simulink model "pfb_fft_d3a"  (R2021a)
settings: Solver=VariableStepAuto  StartTime=0.0  StopTime=100.0  RelTol=1e-3
undefined symbols (not defined in the file): i, pfb_coeff_gen_calc
libraries: xbsIndex_r4 x11529, casper_library_misc x39, casper_library_delays x39, xbsReplacements_r4 x2
(part 2 of 118)

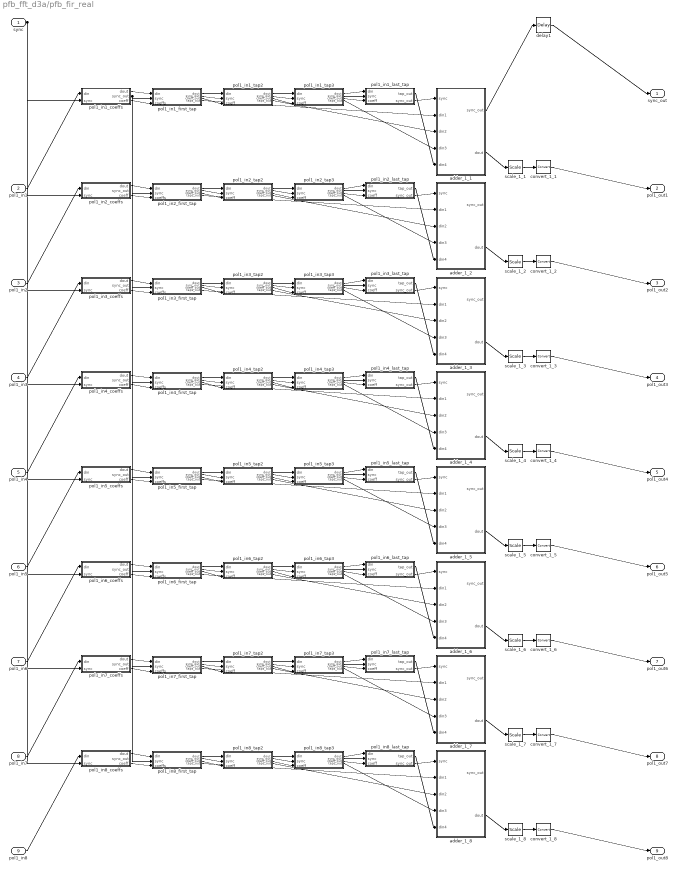
== system pfb_fft_d3a/pfb_fir_real ==
  sync : Inport
  pol1_in1 : Inport  Port=2
  pol1_in2 : Inport  Port=3
  pol1_in3 : Inport  Port=4
  pol1_in4 : Inport  Port=5
  pol1_in5 : Inport  Port=6
  pol1_in6 : Inport  Port=7
  pol1_in7 : Inport  Port=8
  pol1_in8 : Inport  Port=9
  adder_1_1 : Subsystem  AncestorBlock=casper_library_misc/adder_tree  mask(adder_tree){n_inputs=4, csp_latency=1, adder_imp=Fabric, first_stage_hdl=on, floating_point=off, dvalid_en=off, float_type=single, frac_width=0, exp_width=0}
      mask prompts: n_inputs "Number of Inputs"; csp_latency "Add Latency"; adder_imp "Adder implementation"; first_stage_hdl "Use behavioural HDL for first stage of adders"; floating_point "floating point"; float_type "float type"; frac_width "fraction length"; exp_width "exponent length"
      mask help:
      | Sums all inputs using a tree of adds and delays.
      |
      | Number of inputs: The number of inputs to the block to be summed
      | Add latency: The number of clock cycles to perform one addition (affects timing)..
      | Adder implementation: choice of fabric or DSP48E core, or behavioral HDL
      | Use behavioural HDL for first stage of adders: Causes the first stage of adders to be absorbed into DSP blocks if multipliers precede them (Virtex 5). Overrides Adder implementation
      mask init:
      | adder_tree_init(gcb, ...
      |     'n_inputs', n_inputs, ...
      |     'csp_latency', csp_latency, ...
      |     'adder_imp', adder_imp, ...
      |     'dvalid_en', dvalid_en, ...
      |     'floating_point', floating_point, ...
      |     'float_type', float_type, ...
      |     'exp_width', exp_width, ...
      |     'frac_width', frac_width, ...     
      |     'first_stage_hdl', first_stage_hdl);
      settings: AttributesFormatString=latency 2
      mask Help: eval('xlWeb(''http://casper.berkeley.edu/wiki/Adder_tree'')')
      mask TypeOptions adder_imp: Behavioral | Fabric | DSP48
      mask Callback floating_point:
      | onoff = get_param(gcb, 'floating_point');
      | if strcmp(onoff,'on')
      |     enable_fixpt = 'off';
      |     set_param_state(gcb, 'float_type', 'on')
      | 
      |     f_type = get_param(gcb, 'float_type');
      |     if strcmp(f_type,'custom')
      |         set_param_state(gcb, 'exp_width', 'on')
      |         set_param_state(gcb, 'frac_width', 'on')
      |     else
      |         set_param_state(gcb, 'exp_width', 'off')
      |         set_param_state(gcb, 'frac_width', 'off')
      |     end
      | 
      | 
      | else
      |     enable_fixpt = 'on';
      |     set_param_state(gcb, 'float_type', 'off')
      |     set_param_state(gcb, 'exp_width', 'off')
      |     set_param_state(gcb, 'frac_width', 'off')
      | end
      mask TypeOptions float_type: single | custom
      mask Callback float_type:
      | f_type = get_param(gcb, 'float_type');
      | if strcmp(f_type,'custom')
      |     set_param_state(gcb, 'exp_width', 'on')
      |     set_param_state(gcb, 'frac_width', 'on')
      | else
      |     set_param_state(gcb, 'exp_width', 'off')
      |     set_param_state(gcb, 'frac_width', 'off')
      | end
  adder_1_2 : Subsystem  AncestorBlock=casper_library_misc/adder_tree  mask(adder_tree){n_inputs=4, csp_latency=1, adder_imp=Fabric, first_stage_hdl=on, floating_point=off, dvalid_en=off, float_type=single, frac_width=0, exp_width=0}
      mask prompts: n_inputs "Number of Inputs"; csp_latency "Add Latency"; adder_imp "Adder implementation"; first_stage_hdl "Use behavioural HDL for first stage of adders"; floating_point "floating point"; float_type "float type"; frac_width "fraction length"; exp_width "exponent length"
      mask help:
      | Sums all inputs using a tree of adds and delays.
      |
      | Number of inputs: The number of inputs to the block to be summed
      | Add latency: The number of clock cycles to perform one addition (affects timing)..
      | Adder implementation: choice of fabric or DSP48E core, or behavioral HDL
      | Use behavioural HDL for first stage of adders: Causes the first stage of adders to be absorbed into DSP blocks if multipliers precede them (Virtex 5). Overrides Adder implementation
      mask init: same as pfb_fft_d3a/pfb_fir_real/adder_1_1
      settings: AttributesFormatString=latency 2
      mask Help: eval('xlWeb(''http://casper.berkeley.edu/wiki/Adder_tree'')')
      mask TypeOptions adder_imp: Behavioral | Fabric | DSP48
      mask Callback floating_point:
      | onoff = get_param(gcb, 'floating_point');
      | if strcmp(onoff,'on')
      |     enable_fixpt = 'off';
      |     set_param_state(gcb, 'float_type', 'on')
      | 
      |     f_type = get_param(gcb, 'float_type');
      |     if strcmp(f_type,'custom')
      |         set_param_state(gcb, 'exp_width', 'on')
      |         set_param_state(gcb, 'frac_width', 'on')
      |     else
      |         set_param_state(gcb, 'exp_width', 'off')
      |         set_param_state(gcb, 'frac_width', 'off')
      |     end
      | 
      | 
      | else
      |     enable_fixpt = 'on';
      |     set_param_state(gcb, 'float_type', 'off')
      |     set_param_state(gcb, 'exp_width', 'off')
      |     set_param_state(gcb, 'frac_width', 'off')
      | end
      mask TypeOptions float_type: single | custom
      mask Callback float_type:
      | f_type = get_param(gcb, 'float_type');
      | if strcmp(f_type,'custom')
      |     set_param_state(gcb, 'exp_width', 'on')
      |     set_param_state(gcb, 'frac_width', 'on')
      | else
      |     set_param_state(gcb, 'exp_width', 'off')
      |     set_param_state(gcb, 'frac_width', 'off')
      | end
  adder_1_3 : Subsystem  AncestorBlock=casper_library_misc/adder_tree  mask(adder_tree){n_inputs=4, csp_latency=1, adder_imp=Fabric, first_stage_hdl=on, floating_point=off, dvalid_en=off, float_type=single, frac_width=0, exp_width=0}
      mask prompts: n_inputs "Number of Inputs"; csp_latency "Add Latency"; adder_imp "Adder implementation"; first_stage_hdl "Use behavioural HDL for first stage of adders"; floating_point "floating point"; float_type "float type"; frac_width "fraction length"; exp_width "exponent length"
      mask help:
      | Sums all inputs using a tree of adds and delays.
      |
      | Number of inputs: The number of inputs to the block to be summed
      | Add latency: The number of clock cycles to perform one addition (affects timing)..
      | Adder implementation: choice of fabric or DSP48E core, or behavioral HDL
      | Use behavioural HDL for first stage of adders: Causes the first stage of adders to be absorbed into DSP blocks if multipliers precede them (Virtex 5). Overrides Adder implementation
      mask init: same as pfb_fft_d3a/pfb_fir_real/adder_1_1
      settings: AttributesFormatString=latency 2
      mask Help: eval('xlWeb(''http://casper.berkeley.edu/wiki/Adder_tree'')')
      mask TypeOptions adder_imp: Behavioral | Fabric | DSP48
      mask Callback floating_point:
      | onoff = get_param(gcb, 'floating_point');
      | if strcmp(onoff,'on')
      |     enable_fixpt = 'off';
      |     set_param_state(gcb, 'float_type', 'on')
      | 
      |     f_type = get_param(gcb, 'float_type');
      |     if strcmp(f_type,'custom')
      |         set_param_state(gcb, 'exp_width', 'on')
      |         set_param_state(gcb, 'frac_width', 'on')
      |     else
      |         set_param_state(gcb, 'exp_width', 'off')
      |         set_param_state(gcb, 'frac_width', 'off')
      |     end
      | 
      | 
      | else
      |     enable_fixpt = 'on';
      |     set_param_state(gcb, 'float_type', 'off')
      |     set_param_state(gcb, 'exp_width', 'off')
      |     set_param_state(gcb, 'frac_width', 'off')
      | end
      mask TypeOptions float_type: single | custom
      mask Callback float_type:
      | f_type = get_param(gcb, 'float_type');
      | if strcmp(f_type,'custom')
      |     set_param_state(gcb, 'exp_width', 'on')
      |     set_param_state(gcb, 'frac_width', 'on')
      | else
      |     set_param_state(gcb, 'exp_width', 'off')
      |     set_param_state(gcb, 'frac_width', 'off')
      | end
  adder_1_4 : Subsystem  AncestorBlock=casper_library_misc/adder_tree  mask(adder_tree){n_inputs=4, csp_latency=1, adder_imp=Fabric, first_stage_hdl=on, floating_point=off, dvalid_en=off, float_type=single, frac_width=0, exp_width=0}
      mask prompts: n_inputs "Number of Inputs"; csp_latency "Add Latency"; adder_imp "Adder implementation"; first_stage_hdl "Use behavioural HDL for first stage of adders"; floating_point "floating point"; float_type "float type"; frac_width "fraction length"; exp_width "exponent length"
      mask help:
      | Sums all inputs using a tree of adds and delays.
      |
      | Number of inputs: The number of inputs to the block to be summed
      | Add latency: The number of clock cycles to perform one addition (affects timing)..
      | Adder implementation: choice of fabric or DSP48E core, or behavioral HDL
      | Use behavioural HDL for first stage of adders: Causes the first stage of adders to be absorbed into DSP blocks if multipliers precede them (Virtex 5). Overrides Adder implementation
      mask init: same as pfb_fft_d3a/pfb_fir_real/adder_1_1
      settings: AttributesFormatString=latency 2
      mask Help: eval('xlWeb(''http://casper.berkeley.edu/wiki/Adder_tree'')')
      mask TypeOptions adder_imp: Behavioral | Fabric | DSP48
      mask Callback floating_point:
      | onoff = get_param(gcb, 'floating_point');
      | if strcmp(onoff,'on')
      |     enable_fixpt = 'off';
      |     set_param_state(gcb, 'float_type', 'on')
      | 
      |     f_type = get_param(gcb, 'float_type');
      |     if strcmp(f_type,'custom')
      |         set_param_state(gcb, 'exp_width', 'on')
      |         set_param_state(gcb, 'frac_width', 'on')
      |     else
      |         set_param_state(gcb, 'exp_width', 'off')
      |         set_param_state(gcb, 'frac_width', 'off')
      |     end
      | 
      | 
      | else
      |     enable_fixpt = 'on';
      |     set_param_state(gcb, 'float_type', 'off')
      |     set_param_state(gcb, 'exp_width', 'off')
      |     set_param_state(gcb, 'frac_width', 'off')
      | end
      mask TypeOptions float_type: single | custom
      mask Callback float_type:
      | f_type = get_param(gcb, 'float_type');
      | if strcmp(f_type,'custom')
      |     set_param_state(gcb, 'exp_width', 'on')
      |     set_param_state(gcb, 'frac_width', 'on')
      | else
      |     set_param_state(gcb, 'exp_width', 'off')
      |     set_param_state(gcb, 'frac_width', 'off')
      | end
  adder_1_5 : Subsystem  AncestorBlock=casper_library_misc/adder_tree  mask(adder_tree){n_inputs=4, csp_latency=1, adder_imp=Fabric, first_stage_hdl=on, floating_point=off, dvalid_en=off, float_type=single, frac_width=0, exp_width=0}
      mask prompts: n_inputs "Number of Inputs"; csp_latency "Add Latency"; adder_imp "Adder implementation"; first_stage_hdl "Use behavioural HDL for first stage of adders"; floating_point "floating point"; float_type "float type"; frac_width "fraction length"; exp_width "exponent length"
      mask help:
      | Sums all inputs using a tree of adds and delays.
      |
      | Number of inputs: The number of inputs to the block to be summed
      | Add latency: The number of clock cycles to perform one addition (affects timing)..
      | Adder implementation: choice of fabric or DSP48E core, or behavioral HDL
      | Use behavioural HDL for first stage of adders: Causes the first stage of adders to be absorbed into DSP blocks if multipliers precede them (Virtex 5). Overrides Adder implementation
      mask init: same as pfb_fft_d3a/pfb_fir_real/adder_1_1
      settings: AttributesFormatString=latency 2
      mask Help: eval('xlWeb(''http://casper.berkeley.edu/wiki/Adder_tree'')')
      mask TypeOptions adder_imp: Behavioral | Fabric | DSP48
      mask Callback floating_point:
      | onoff = get_param(gcb, 'floating_point');
      | if strcmp(onoff,'on')
      |     enable_fixpt = 'off';
      |     set_param_state(gcb, 'float_type', 'on')
      | 
      |     f_type = get_param(gcb, 'float_type');
      |     if strcmp(f_type,'custom')
      |         set_param_state(gcb, 'exp_width', 'on')
      |         set_param_state(gcb, 'frac_width', 'on')
      |     else
      |         set_param_state(gcb, 'exp_width', 'off')
      |         set_param_state(gcb, 'frac_width', 'off')
      |     end
      | 
      | 
      | else
      |     enable_fixpt = 'on';
      |     set_param_state(gcb, 'float_type', 'off')
      |     set_param_state(gcb, 'exp_width', 'off')
      |     set_param_state(gcb, 'frac_width', 'off')
      | end
      mask TypeOptions float_type: single | custom
      mask Callback float_type:
      | f_type = get_param(gcb, 'float_type');
      | if strcmp(f_type,'custom')
      |     set_param_state(gcb, 'exp_width', 'on')
      |     set_param_state(gcb, 'frac_width', 'on')
      | else
      |     set_param_state(gcb, 'exp_width', 'off')
      |     set_param_state(gcb, 'frac_width', 'off')
      | end
  adder_1_6 : Subsystem  AncestorBlock=casper_library_misc/adder_tree  mask(adder_tree){n_inputs=4, csp_latency=1, adder_imp=Fabric, first_stage_hdl=on, floating_point=off, dvalid_en=off, float_type=single, frac_width=0, exp_width=0}
      mask prompts: n_inputs "Number of Inputs"; csp_latency "Add Latency"; adder_imp "Adder implementation"; first_stage_hdl "Use behavioural HDL for first stage of adders"; floating_point "floating point"; float_type "float type"; frac_width "fraction length"; exp_width "exponent length"
      mask help:
      | Sums all inputs using a tree of adds and delays.
      |
      | Number of inputs: The number of inputs to the block to be summed
      | Add latency: The number of clock cycles to perform one addition (affects timing)..
      | Adder implementation: choice of fabric or DSP48E core, or behavioral HDL
      | Use behavioural HDL for first stage of adders: Causes the first stage of adders to be absorbed into DSP blocks if multipliers precede them (Virtex 5). Overrides Adder implementation
      mask init: same as pfb_fft_d3a/pfb_fir_real/adder_1_1
      settings: AttributesFormatString=latency 2
      mask Help: eval('xlWeb(''http://casper.berkeley.edu/wiki/Adder_tree'')')
      mask TypeOptions adder_imp: Behavioral | Fabric | DSP48
      mask Callback floating_point:
      | onoff = get_param(gcb, 'floating_point');
      | if strcmp(onoff,'on')
      |     enable_fixpt = 'off';
      |     set_param_state(gcb, 'float_type', 'on')
      | 
      |     f_type = get_param(gcb, 'float_type');
      |     if strcmp(f_type,'custom')
      |         set_param_state(gcb, 'exp_width', 'on')
      |         set_param_state(gcb, 'frac_width', 'on')
      |     else
      |         set_param_state(gcb, 'exp_width', 'off')
      |         set_param_state(gcb, 'frac_width', 'off')
      |     end
      | 
      | 
      | else
      |     enable_fixpt = 'on';
      |     set_param_state(gcb, 'float_type', 'off')
      |     set_param_state(gcb, 'exp_width', 'off')
      |     set_param_state(gcb, 'frac_width', 'off')
      | end
      mask TypeOptions float_type: single | custom
      mask Callback float_type:
      | f_type = get_param(gcb, 'float_type');
      | if strcmp(f_type,'custom')
      |     set_param_state(gcb, 'exp_width', 'on')
      |     set_param_state(gcb, 'frac_width', 'on')
      | else
      |     set_param_state(gcb, 'exp_width', 'off')
      |     set_param_state(gcb, 'frac_width', 'off')
      | end
  adder_1_7 : Subsystem  AncestorBlock=casper_library_misc/adder_tree  mask(adder_tree){n_inputs=4, csp_latency=1, adder_imp=Fabric, first_stage_hdl=on, floating_point=off, dvalid_en=off, float_type=single, frac_width=0, exp_width=0}
      mask prompts: n_inputs "Number of Inputs"; csp_latency "Add Latency"; adder_imp "Adder implementation"; first_stage_hdl "Use behavioural HDL for first stage of adders"; floating_point "floating point"; float_type "float type"; frac_width "fraction length"; exp_width "exponent length"
      mask help:
      | Sums all inputs using a tree of adds and delays.
      |
      | Number of inputs: The number of inputs to the block to be summed
      | Add latency: The number of clock cycles to perform one addition (affects timing)..
      | Adder implementation: choice of fabric or DSP48E core, or behavioral HDL
      | Use behavioural HDL for first stage of adders: Causes the first stage of adders to be absorbed into DSP blocks if multipliers precede them (Virtex 5). Overrides Adder implementation
      mask init: same as pfb_fft_d3a/pfb_fir_real/adder_1_1
      settings: AttributesFormatString=latency 2
      mask Help: eval('xlWeb(''http://casper.berkeley.edu/wiki/Adder_tree'')')
      mask TypeOptions adder_imp: Behavioral | Fabric | DSP48
      mask Callback floating_point:
      | onoff = get_param(gcb, 'floating_point');
      | if strcmp(onoff,'on')
      |     enable_fixpt = 'off';
      |     set_param_state(gcb, 'float_type', 'on')
      | 
      |     f_type = get_param(gcb, 'float_type');
      |     if strcmp(f_type,'custom')
      |         set_param_state(gcb, 'exp_width', 'on')
      |         set_param_state(gcb, 'frac_width', 'on')
      |     else
      |         set_param_state(gcb, 'exp_width', 'off')
      |         set_param_state(gcb, 'frac_width', 'off')
      |     end
      | 
      | 
      | else
      |     enable_fixpt = 'on';
      |     set_param_state(gcb, 'float_type', 'off')
      |     set_param_state(gcb, 'exp_width', 'off')
      |     set_param_state(gcb, 'frac_width', 'off')
      | end
      mask TypeOptions float_type: single | custom
      mask Callback float_type:
      | f_type = get_param(gcb, 'float_type');
      | if strcmp(f_type,'custom')
      |     set_param_state(gcb, 'exp_width', 'on')
      |     set_param_state(gcb, 'frac_width', 'on')
      | else
      |     set_param_state(gcb, 'exp_width', 'off')
      |     set_param_state(gcb, 'frac_width', 'off')
      | end
  adder_1_8 : Subsystem  AncestorBlock=casper_library_misc/adder_tree  mask(adder_tree){n_inputs=4, csp_latency=1, adder_imp=Fabric, first_stage_hdl=on, floating_point=off, dvalid_en=off, float_type=single, frac_width=0, exp_width=0}
      mask prompts: n_inputs "Number of Inputs"; csp_latency "Add Latency"; adder_imp "Adder implementation"; first_stage_hdl "Use behavioural HDL for first stage of adders"; floating_point "floating point"; float_type "float type"; frac_width "fraction length"; exp_width "exponent length"
      mask help:
      | Sums all inputs using a tree of adds and delays.
      |
      | Number of inputs: The number of inputs to the block to be summed
      | Add latency: The number of clock cycles to perform one addition (affects timing)..
      | Adder implementation: choice of fabric or DSP48E core, or behavioral HDL
      | Use behavioural HDL for first stage of adders: Causes the first stage of adders to be absorbed into DSP blocks if multipliers precede them (Virtex 5). Overrides Adder implementation
      mask init: same as pfb_fft_d3a/pfb_fir_real/adder_1_1
      settings: AttributesFormatString=latency 2
      mask Help: eval('xlWeb(''http://casper.berkeley.edu/wiki/Adder_tree'')')
      mask TypeOptions adder_imp: Behavioral | Fabric | DSP48
      mask Callback floating_point:
      | onoff = get_param(gcb, 'floating_point');
      | if strcmp(onoff,'on')
      |     enable_fixpt = 'off';
      |     set_param_state(gcb, 'float_type', 'on')
      | 
      |     f_type = get_param(gcb, 'float_type');
      |     if strcmp(f_type,'custom')
      |         set_param_state(gcb, 'exp_width', 'on')
      |         set_param_state(gcb, 'frac_width', 'on')
      |     else
      |         set_param_state(gcb, 'exp_width', 'off')
      |         set_param_state(gcb, 'frac_width', 'off')
      |     end
      | 
      | 
      | else
      |     enable_fixpt = 'on';
      |     set_param_state(gcb, 'float_type', 'off')
      |     set_param_state(gcb, 'exp_width', 'off')
      |     set_param_state(gcb, 'frac_width', 'off')
      | end
      mask TypeOptions float_type: single | custom
      mask Callback float_type:
      | f_type = get_param(gcb, 'float_type');
      | if strcmp(f_type,'custom')
      |     set_param_state(gcb, 'exp_width', 'on')
      |     set_param_state(gcb, 'frac_width', 'on')
      | else
      |     set_param_state(gcb, 'exp_width', 'off')
      |     set_param_state(gcb, 'frac_width', 'off')
      | end
  convert_1_{1..8} (8 alike) : xbsIndex_r4/Convert  gui_display_data_type=Fixed-point  arith_type="Signed  (2's comp)"  n_bits=18  bin_pt=17  float_type=Single  exp_bits=8  fraction_bits=24  quantization="Round  (unbiased: Even Values)"  overflow=Wrap  en=off  latency=1  pipeline=on  dbl_ovrd=off  block_type=convert
  delay1 : xbsIndex_r4/Delay  rst=off  infoeditControl=Selection of Reset will increase slice count due to use of real FFs and instead of SRLs  en=off  latency=1  reg_retiming=off  dbl_ovrd=off  block_type=delay
  pol1_in1_coeffs : Subsystem  AncestorBlock=casper_library_pfbs/pfb_coeff_gen  mask(pfb_coeff_gen){PFBSize=14, CoeffBitWidth=18, TotalTaps=4, CoeffDistMem=off, WindowType=hamming, bram_latency=2, n_inputs=3, nput=0, fwidth=1, debug_mode=off, fan_latency=1}
      mask prompts: PFBSize "Size of PFB: (2^? pnts)"; CoeffBitWidth "Bitwidth of Coefficients:"; TotalTaps "Total Number of Taps:"; CoeffDistMem "Implement Coeff Gen in Distributed Memory"; WindowType "Windowing Function:"; bram_latency "BRAM Latency"; n_inputs "Number of Simultaneous Inputs: (2^?)"; nput "This is input number:"; fwidth "Bin Width (normal=1)"; debug_mode "Debug mode - coeffs are a [1:pfb_size*taps] ramp."; fan_latency "Fanout latency"
      mask init:
      | pfb_coeff_gen_init(gcb, ...
      |     'PFBSize', PFBSize, ...
      |     'CoeffBitWidth', CoeffBitWidth, ...
      |     'TotalTaps', TotalTaps, ...
      |     'CoeffDistMem', CoeffDistMem, ...
      |     'WindowType', WindowType, ...
      |     'bram_latency', bram_latency, ...
      |     'n_inputs', n_inputs, ...
      |     'nput', nput, ...
      |     'fwidth', fwidth, ...
      |     'fan_latency', fan_latency, ...
      |     'debug_mode', debug_mode);
      settings: AttributesFormatString=|
      | PFBSize=14, n_inputs=3,
      | taps=4, input=0
  pol1_in1_first_tap : Subsystem  AncestorBlock=casper_library_pfbs/first_tap_real  mask(first_tap_real){PFBSize=14, n_pol_blocks=1, CoeffBitWidth=18, TotalTaps=4, BitWidthIn=14, WindowType=hamming, mult_latency=2, bram_latency=2, n_inputs=3, fwidth=1, use_hdl=on, use_embedded=off}
      mask prompts: PFBSize "Size of PFB: (2^? pnts)"; n_pol_blocks "Number of serial polarization blocks"; CoeffBitWidth "Bitwidth of Coefficients:"; TotalTaps "Total Number of Taps:"; BitWidthIn "Input Bitwidth:"; WindowType "Windowing Function:"; mult_latency "Mult Latency"; bram_latency "BRAM Latency"; n_inputs "Number of Simultaneous Inputs: (2^?)"; fwidth "Bit Width (normal=1)"; use_hdl "Use behavioral HDL for multlipliers"; use_embedded "Use embedded multipliers"
      mask init:
      | first_tap_real_init(gcb,...
      |     'PFBSize', PFBSize,...
      |     'CoeffBitWidth', CoeffBitWidth,...
      |     'TotalTaps', TotalTaps,...
      |     'BitWidthIn', BitWidthIn,...
      |     'WindowType', WindowType,...
      |     'mult_latency', mult_latency,...
      |     'bram_latency', bram_latency,...
      |     'n_inputs', n_inputs,...
      |     'n_pol_blocks', n_pol_blocks, ...
      |     'fwidth', fwidth,...
      |     'use_hdl', use_hdl,...
      |     'use_embedded', use_embedded);
      settings: AttributesFormatString=taps=4
      mask TypeOptions WindowType: bartlett | barthannwin | blackman | blackmanharris | bohamwin | chebwin | flattopwin | gausswin | hamming | hann | kaiser | nuttallwin | parzenwin | rectwin | tukeywin | triang | userwindow
      mask Callback use_hdl:
      | use_hdl = get_param(gcb,'use_hdl');
      | if( strcmp(use_hdl,'on')),
      |     set_param(gcb, 'use_embedded','off');
      |     set_param(gcb, 'MaskVisibilities',{'on','on','on','on','on','on','on','on','on','on','on','off'});
      | else,
      |     set_param(gcb, 'MaskVisibilities',{'on','on','on','on','on','on','on','on','on','on','on','on'});
      | end
  pol1_in1_last_tap : Subsystem  AncestorBlock=casper_library_pfbs/last_tap_real  mask(last_tap_real){BitWidthIn=14, CoeffBitWidth=18, mult_latency=2, use_hdl=on, use_embedded=off}
      mask prompts: BitWidthIn "Input Bitwidth:"; CoeffBitWidth "Coeff Bitwidth:"; mult_latency "Mult Latency"; use_hdl "Use behavioral HDL for multlipliers"; use_embedded "Use embedded multipliers"
      mask init:
      | last_tap_real_init(gcb,...
      |     'BitWidthIn', BitWidthIn,...
      |     'CoeffBitWidth', CoeffBitWidth,...
      |     'mult_latency', mult_latency,...
      |     'use_hdl', use_hdl,...
      |     'use_embedded', use_embedded);
      mask Callback use_hdl:
      | use_hdl = get_param(gcb,'use_hdl');
      | if( strcmp(use_hdl,'on')),
      |     set_param(gcb, 'use_embedded','off');
      |     set_param(gcb, 'MaskVisibilities',{'on','on','on','on','off'});
      | else,
      |     set_param(gcb, 'MaskVisibilities',{'on','on','on','on','on'});
      | end
  pol1_in1_tap2 : Subsystem  AncestorBlock=casper_library_pfbs/tap_real  mask(pfb_tap_real){mult_latency=2, coeff_width=18, coeff_frac_width=17, delay=2048, data_width=14, bram_latency=2, use_hdl=on, use_embedded=off}
      mask prompts: mult_latency "Multiplier Latency"; coeff_width "Coefficient Bit Width In"; coeff_frac_width "Coefficient Fractional Bits"; delay "Data/Sync Delay"; data_width "Data Bit Width In"; bram_latency "BRAM Latency"; use_hdl "Use behavioral HDL for multlipliers"; use_embedded "Use embedded multipliers"
      mask init:
      | use_hdl = get_param(gcb,'use_hdl');
      | use_embedded = get_param(gcb,'use_embedded');
      | set_param(gcb,'LinkStatus','inactive');
      | 
      | set_param([gcb,'/Mult'],'use_embedded',use_embedded);
      | set_param([gcb,'/Mult'],'use_behavioral_HDL',use_hdl);
  pol1_in1_tap3 : Subsystem  AncestorBlock=casper_library_pfbs/tap_real  mask(pfb_tap_real){mult_latency=2, coeff_width=18, coeff_frac_width=17, delay=2048, data_width=14, bram_latency=2, use_hdl=on, use_embedded=off}
      mask prompts: mult_latency "Multiplier Latency"; coeff_width "Coefficient Bit Width In"; coeff_frac_width "Coefficient Fractional Bits"; delay "Data/Sync Delay"; data_width "Data Bit Width In"; bram_latency "BRAM Latency"; use_hdl "Use behavioral HDL for multlipliers"; use_embedded "Use embedded multipliers"
      mask init: same as pfb_fft_d3a/pfb_fir_real/pol1_in1_tap2
  pol1_in2_coeffs : Subsystem  AncestorBlock=casper_library_pfbs/pfb_coeff_gen  mask(pfb_coeff_gen){PFBSize=14, CoeffBitWidth=18, TotalTaps=4, CoeffDistMem=off, WindowType=hamming, bram_latency=2, n_inputs=3, nput=1, fwidth=1, debug_mode=off, fan_latency=1}
      mask prompts: PFBSize "Size of PFB: (2^? pnts)"; CoeffBitWidth "Bitwidth of Coefficients:"; TotalTaps "Total Number of Taps:"; CoeffDistMem "Implement Coeff Gen in Distributed Memory"; WindowType "Windowing Function:"; bram_latency "BRAM Latency"; n_inputs "Number of Simultaneous Inputs: (2^?)"; nput "This is input number:"; fwidth "Bin Width (normal=1)"; debug_mode "Debug mode - coeffs are a [1:pfb_size*taps] ramp."; fan_latency "Fanout latency"
      mask init: same as pfb_fft_d3a/pfb_fir_real/pol1_in1_coeffs
      settings: AttributesFormatString=|
      | PFBSize=14, n_inputs=3,
      | taps=4, input=1
  pol1_in2_first_tap : Subsystem  AncestorBlock=casper_library_pfbs/first_tap_real  mask(first_tap_real){PFBSize=14, n_pol_blocks=1, CoeffBitWidth=18, TotalTaps=4, BitWidthIn=14, WindowType=hamming, mult_latency=2, bram_latency=2, n_inputs=3, fwidth=1, use_hdl=on, use_embedded=off}
      mask prompts: PFBSize "Size of PFB: (2^? pnts)"; n_pol_blocks "Number of serial polarization blocks"; CoeffBitWidth "Bitwidth of Coefficients:"; TotalTaps "Total Number of Taps:"; BitWidthIn "Input Bitwidth:"; WindowType "Windowing Function:"; mult_latency "Mult Latency"; bram_latency "BRAM Latency"; n_inputs "Number of Simultaneous Inputs: (2^?)"; fwidth "Bit Width (normal=1)"; use_hdl "Use behavioral HDL for multlipliers"; use_embedded "Use embedded multipliers"
      mask init: same as pfb_fft_d3a/pfb_fir_real/pol1_in1_first_tap
      settings: AttributesFormatString=taps=4
      mask TypeOptions WindowType: bartlett | barthannwin | blackman | blackmanharris | bohamwin | chebwin | flattopwin | gausswin | hamming | hann | kaiser | nuttallwin | parzenwin | rectwin | tukeywin | triang | userwindow
      mask Callback use_hdl:
      | use_hdl = get_param(gcb,'use_hdl');
      | if( strcmp(use_hdl,'on')),
      |     set_param(gcb, 'use_embedded','off');
      |     set_param(gcb, 'MaskVisibilities',{'on','on','on','on','on','on','on','on','on','on','on','off'});
      | else,
      |     set_param(gcb, 'MaskVisibilities',{'on','on','on','on','on','on','on','on','on','on','on','on'});
      | end
  pol1_in2_last_tap : Subsystem  AncestorBlock=casper_library_pfbs/last_tap_real  mask(last_tap_real){BitWidthIn=14, CoeffBitWidth=18, mult_latency=2, use_hdl=on, use_embedded=off}
      mask prompts: BitWidthIn "Input Bitwidth:"; CoeffBitWidth "Coeff Bitwidth:"; mult_latency "Mult Latency"; use_hdl "Use behavioral HDL for multlipliers"; use_embedded "Use embedded multipliers"
      mask init:
      | last_tap_real_init(gcb,...
      |     'BitWidthIn', BitWidthIn,...
      |     'CoeffBitWidth', CoeffBitWidth,...
      |     'mult_latency', mult_latency,...
      |     'use_hdl', use_hdl,...
      |     'use_embedded', use_embedded);
      mask Callback use_hdl:
      | use_hdl = get_param(gcb,'use_hdl');
      | if( strcmp(use_hdl,'on')),
      |     set_param(gcb, 'use_embedded','off');
      |     set_param(gcb, 'MaskVisibilities',{'on','on','on','on','off'});
      | else,
      |     set_param(gcb, 'MaskVisibilities',{'on','on','on','on','on'});
      | end
  pol1_in2_tap2 : Subsystem  AncestorBlock=casper_library_pfbs/tap_real  mask(pfb_tap_real){mult_latency=2, coeff_width=18, coeff_frac_width=17, delay=2048, data_width=14, bram_latency=2, use_hdl=on, use_embedded=off}
      mask prompts: mult_latency "Multiplier Latency"; coeff_width "Coefficient Bit Width In"; coeff_frac_width "Coefficient Fractional Bits"; delay "Data/Sync Delay"; data_width "Data Bit Width In"; bram_latency "BRAM Latency"; use_hdl "Use behavioral HDL for multlipliers"; use_embedded "Use embedded multipliers"
      mask init: same as pfb_fft_d3a/pfb_fir_real/pol1_in1_tap2
  pol1_in2_tap3 : Subsystem  AncestorBlock=casper_library_pfbs/tap_real  mask(pfb_tap_real){mult_latency=2, coeff_width=18, coeff_frac_width=17, delay=2048, data_width=14, bram_latency=2, use_hdl=on, use_embedded=off}
      mask prompts: mult_latency "Multiplier Latency"; coeff_width "Coefficient Bit Width In"; coeff_frac_width "Coefficient Fractional Bits"; delay "Data/Sync Delay"; data_width "Data Bit Width In"; bram_latency "BRAM Latency"; use_hdl "Use behavioral HDL for multlipliers"; use_embedded "Use embedded multipliers"
      mask init: same as pfb_fft_d3a/pfb_fir_real/pol1_in1_tap2
  pol1_in3_coeffs : Subsystem  AncestorBlock=casper_library_pfbs/pfb_coeff_gen  mask(pfb_coeff_gen){PFBSize=14, CoeffBitWidth=18, TotalTaps=4, CoeffDistMem=off, WindowType=hamming, bram_latency=2, n_inputs=3, nput=2, fwidth=1, debug_mode=off, fan_latency=1}
      mask prompts: PFBSize "Size of PFB: (2^? pnts)"; CoeffBitWidth "Bitwidth of Coefficients:"; TotalTaps "Total Number of Taps:"; CoeffDistMem "Implement Coeff Gen in Distributed Memory"; WindowType "Windowing Function:"; bram_latency "BRAM Latency"; n_inputs "Number of Simultaneous Inputs: (2^?)"; nput "This is input number:"; fwidth "Bin Width (normal=1)"; debug_mode "Debug mode - coeffs are a [1:pfb_size*taps] ramp."; fan_latency "Fanout latency"
      mask init: same as pfb_fft_d3a/pfb_fir_real/pol1_in1_coeffs
      settings: AttributesFormatString=|
      | PFBSize=14, n_inputs=3,
      | taps=4, input=2
  pol1_in3_first_tap : Subsystem  AncestorBlock=casper_library_pfbs/first_tap_real  mask(first_tap_real){PFBSize=14, n_pol_blocks=1, CoeffBitWidth=18, TotalTaps=4, BitWidthIn=14, WindowType=hamming, mult_latency=2, bram_latency=2, n_inputs=3, fwidth=1, use_hdl=on, use_embedded=off}
      mask prompts: PFBSize "Size of PFB: (2^? pnts)"; n_pol_blocks "Number of serial polarization blocks"; CoeffBitWidth "Bitwidth of Coefficients:"; TotalTaps "Total Number of Taps:"; BitWidthIn "Input Bitwidth:"; WindowType "Windowing Function:"; mult_latency "Mult Latency"; bram_latency "BRAM Latency"; n_inputs "Number of Simultaneous Inputs: (2^?)"; fwidth "Bit Width (normal=1)"; use_hdl "Use behavioral HDL for multlipliers"; use_embedded "Use embedded multipliers"
      mask init: same as pfb_fft_d3a/pfb_fir_real/pol1_in1_first_tap
      settings: AttributesFormatString=taps=4
      mask TypeOptions WindowType: bartlett | barthannwin | blackman | blackmanharris | bohamwin | chebwin | flattopwin | gausswin | hamming | hann | kaiser | nuttallwin | parzenwin | rectwin | tukeywin | triang | userwindow
      mask Callback use_hdl:
      | use_hdl = get_param(gcb,'use_hdl');
      | if( strcmp(use_hdl,'on')),
      |     set_param(gcb, 'use_embedded','off');
      |     set_param(gcb, 'MaskVisibilities',{'on','on','on','on','on','on','on','on','on','on','on','off'});
      | else,
      |     set_param(gcb, 'MaskVisibilities',{'on','on','on','on','on','on','on','on','on','on','on','on'});
      | end
  pol1_in3_last_tap : Subsystem  AncestorBlock=casper_library_pfbs/last_tap_real  mask(last_tap_real){BitWidthIn=14, CoeffBitWidth=18, mult_latency=2, use_hdl=on, use_embedded=off}
      mask prompts: BitWidthIn "Input Bitwidth:"; CoeffBitWidth "Coeff Bitwidth:"; mult_latency "Mult Latency"; use_hdl "Use behavioral HDL for multlipliers"; use_embedded "Use embedded multipliers"
      mask init:
      | last_tap_real_init(gcb,...
      |     'BitWidthIn', BitWidthIn,...
      |     'CoeffBitWidth', CoeffBitWidth,...
      |     'mult_latency', mult_latency,...
      |     'use_hdl', use_hdl,...
      |     'use_embedded', use_embedded);
      mask Callback use_hdl:
      | use_hdl = get_param(gcb,'use_hdl');
      | if( strcmp(use_hdl,'on')),
      |     set_param(gcb, 'use_embedded','off');
      |     set_param(gcb, 'MaskVisibilities',{'on','on','on','on','off'});
      | else,
      |     set_param(gcb, 'MaskVisibilities',{'on','on','on','on','on'});
      | end
  pol1_in3_tap2 : Subsystem  AncestorBlock=casper_library_pfbs/tap_real  mask(pfb_tap_real){mult_latency=2, coeff_width=18, coeff_frac_width=17, delay=2048, data_width=14, bram_latency=2, use_hdl=on, use_embedded=off}
      mask prompts: mult_latency "Multiplier Latency"; coeff_width "Coefficient Bit Width In"; coeff_frac_width "Coefficient Fractional Bits"; delay "Data/Sync Delay"; data_width "Data Bit Width In"; bram_latency "BRAM Latency"; use_hdl "Use behavioral HDL for multlipliers"; use_embedded "Use embedded multipliers"
      mask init: same as pfb_fft_d3a/pfb_fir_real/pol1_in1_tap2
  pol1_in3_tap3 : Subsystem  AncestorBlock=casper_library_pfbs/tap_real  mask(pfb_tap_real){mult_latency=2, coeff_width=18, coeff_frac_width=17, delay=2048, data_width=14, bram_latency=2, use_hdl=on, use_embedded=off}
      mask prompts: mult_latency "Multiplier Latency"; coeff_width "Coefficient Bit Width In"; coeff_frac_width "Coefficient Fractional Bits"; delay "Data/Sync Delay"; data_width "Data Bit Width In"; bram_latency "BRAM Latency"; use_hdl "Use behavioral HDL for multlipliers"; use_embedded "Use embedded multipliers"
      mask init: same as pfb_fft_d3a/pfb_fir_real/pol1_in1_tap2
  pol1_in4_coeffs : Subsystem  AncestorBlock=casper_library_pfbs/pfb_coeff_gen  mask(pfb_coeff_gen){PFBSize=14, CoeffBitWidth=18, TotalTaps=4, CoeffDistMem=off, WindowType=hamming, bram_latency=2, n_inputs=3, nput=3, fwidth=1, debug_mode=off, fan_latency=1}
      mask prompts: PFBSize "Size of PFB: (2^? pnts)"; CoeffBitWidth "Bitwidth of Coefficients:"; TotalTaps "Total Number of Taps:"; CoeffDistMem "Implement Coeff Gen in Distributed Memory"; WindowType "Windowing Function:"; bram_latency "BRAM Latency"; n_inputs "Number of Simultaneous Inputs: (2^?)"; nput "This is input number:"; fwidth "Bin Width (normal=1)"; debug_mode "Debug mode - coeffs are a [1:pfb_size*taps] ramp."; fan_latency "Fanout latency"
      mask init: same as pfb_fft_d3a/pfb_fir_real/pol1_in1_coeffs
      settings: AttributesFormatString=|
      | PFBSize=14, n_inputs=3,
      | taps=4, input=3
  pol1_in4_first_tap : Subsystem  AncestorBlock=casper_library_pfbs/first_tap_real  mask(first_tap_real){PFBSize=14, n_pol_blocks=1, CoeffBitWidth=18, TotalTaps=4, BitWidthIn=14, WindowType=hamming, mult_latency=2, bram_latency=2, n_inputs=3, fwidth=1, use_hdl=on, use_embedded=off}
      mask prompts: PFBSize "Size of PFB: (2^? pnts)"; n_pol_blocks "Number of serial polarization blocks"; CoeffBitWidth "Bitwidth of Coefficients:"; TotalTaps "Total Number of Taps:"; BitWidthIn "Input Bitwidth:"; WindowType "Windowing Function:"; mult_latency "Mult Latency"; bram_latency "BRAM Latency"; n_inputs "Number of Simultaneous Inputs: (2^?)"; fwidth "Bit Width (normal=1)"; use_hdl "Use behavioral HDL for multlipliers"; use_embedded "Use embedded multipliers"
      mask init: same as pfb_fft_d3a/pfb_fir_real/pol1_in1_first_tap
      settings: AttributesFormatString=taps=4
      mask TypeOptions WindowType: bartlett | barthannwin | blackman | blackmanharris | bohamwin | chebwin | flattopwin | gausswin | hamming | hann | kaiser | nuttallwin | parzenwin | rectwin | tukeywin | triang | userwindow
      mask Callback use_hdl:
      | use_hdl = get_param(gcb,'use_hdl');
      | if( strcmp(use_hdl,'on')),
      |     set_param(gcb, 'use_embedded','off');
      |     set_param(gcb, 'MaskVisibilities',{'on','on','on','on','on','on','on','on','on','on','on','off'});
      | else,
      |     set_param(gcb, 'MaskVisibilities',{'on','on','on','on','on','on','on','on','on','on','on','on'});
      | end
  pol1_in4_last_tap : Subsystem  AncestorBlock=casper_library_pfbs/last_tap_real  mask(last_tap_real){BitWidthIn=14, CoeffBitWidth=18, mult_latency=2, use_hdl=on, use_embedded=off}
      mask prompts: BitWidthIn "Input Bitwidth:"; CoeffBitWidth "Coeff Bitwidth:"; mult_latency "Mult Latency"; use_hdl "Use behavioral HDL for multlipliers"; use_embedded "Use embedded multipliers"
      mask init:
      | last_tap_real_init(gcb,...
      |     'BitWidthIn', BitWidthIn,...
      |     'CoeffBitWidth', CoeffBitWidth,...
      |     'mult_latency', mult_latency,...
      |     'use_hdl', use_hdl,...
      |     'use_embedded', use_embedded);
      mask Callback use_hdl:
      | use_hdl = get_param(gcb,'use_hdl');
      | if( strcmp(use_hdl,'on')),
      |     set_param(gcb, 'use_embedded','off');
      |     set_param(gcb, 'MaskVisibilities',{'on','on','on','on','off'});
      | else,
      |     set_param(gcb, 'MaskVisibilities',{'on','on','on','on','on'});
      | end
  pol1_in4_tap2 : Subsystem  AncestorBlock=casper_library_pfbs/tap_real  mask(pfb_tap_real){mult_latency=2, coeff_width=18, coeff_frac_width=17, delay=2048, data_width=14, bram_latency=2, use_hdl=on, use_embedded=off}
      mask prompts: mult_latency "Multiplier Latency"; coeff_width "Coefficient Bit Width In"; coeff_frac_width "Coefficient Fractional Bits"; delay "Data/Sync Delay"; data_width "Data Bit Width In"; bram_latency "BRAM Latency"; use_hdl "Use behavioral HDL for multlipliers"; use_embedded "Use embedded multipliers"
      mask init: same as pfb_fft_d3a/pfb_fir_real/pol1_in1_tap2
  pol1_in4_tap3 : Subsystem  AncestorBlock=casper_library_pfbs/tap_real  mask(pfb_tap_real){mult_latency=2, coeff_width=18, coeff_frac_width=17, delay=2048, data_width=14, bram_latency=2, use_hdl=on, use_embedded=off}
      mask prompts: mult_latency "Multiplier Latency"; coeff_width "Coefficient Bit Width In"; coeff_frac_width "Coefficient Fractional Bits"; delay "Data/Sync Delay"; data_width "Data Bit Width In"; bram_latency "BRAM Latency"; use_hdl "Use behavioral HDL for multlipliers"; use_embedded "Use embedded multipliers"
      mask init: same as pfb_fft_d3a/pfb_fir_real/pol1_in1_tap2
  pol1_in5_coeffs : Subsystem  AncestorBlock=casper_library_pfbs/pfb_coeff_gen  mask(pfb_coeff_gen){PFBSize=14, CoeffBitWidth=18, TotalTaps=4, CoeffDistMem=off, WindowType=hamming, bram_latency=2, n_inputs=3, nput=4, fwidth=1, debug_mode=off, fan_latency=1}
      mask prompts: PFBSize "Size of PFB: (2^? pnts)"; CoeffBitWidth "Bitwidth of Coefficients:"; TotalTaps "Total Number of Taps:"; CoeffDistMem "Implement Coeff Gen in Distributed Memory"; WindowType "Windowing Function:"; bram_latency "BRAM Latency"; n_inputs "Number of Simultaneous Inputs: (2^?)"; nput "This is input number:"; fwidth "Bin Width (normal=1)"; debug_mode "Debug mode - coeffs are a [1:pfb_size*taps] ramp."; fan_latency "Fanout latency"
      mask init: same as pfb_fft_d3a/pfb_fir_real/pol1_in1_coeffs
      settings: AttributesFormatString=|
      | PFBSize=14, n_inputs=3,
      | taps=4, input=4
  pol1_in5_first_tap : Subsystem  AncestorBlock=casper_library_pfbs/first_tap_real  mask(first_tap_real){PFBSize=14, n_pol_blocks=1, CoeffBitWidth=18, TotalTaps=4, BitWidthIn=14, WindowType=hamming, mult_latency=2, bram_latency=2, n_inputs=3, fwidth=1, use_hdl=on, use_embedded=off}
      mask prompts: PFBSize "Size of PFB: (2^? pnts)"; n_pol_blocks "Number of serial polarization blocks"; CoeffBitWidth "Bitwidth of Coefficients:"; TotalTaps "Total Number of Taps:"; BitWidthIn "Input Bitwidth:"; WindowType "Windowing Function:"; mult_latency "Mult Latency"; bram_latency "BRAM Latency"; n_inputs "Number of Simultaneous Inputs: (2^?)"; fwidth "Bit Width (normal=1)"; use_hdl "Use behavioral HDL for multlipliers"; use_embedded "Use embedded multipliers"
      mask init: same as pfb_fft_d3a/pfb_fir_real/pol1_in1_first_tap
      settings: AttributesFormatString=taps=4
      mask TypeOptions WindowType: bartlett | barthannwin | blackman | blackmanharris | bohamwin | chebwin | flattopwin | gausswin | hamming | hann | kaiser | nuttallwin | parzenwin | rectwin | tukeywin | triang | userwindow
      mask Callback use_hdl:
      | use_hdl = get_param(gcb,'use_hdl');
      | if( strcmp(use_hdl,'on')),
      |     set_param(gcb, 'use_embedded','off');
      |     set_param(gcb, 'MaskVisibilities',{'on','on','on','on','on','on','on','on','on','on','on','off'});
      | else,
      |     set_param(gcb, 'MaskVisibilities',{'on','on','on','on','on','on','on','on','on','on','on','on'});
      | end
  pol1_in5_last_tap : Subsystem  AncestorBlock=casper_library_pfbs/last_tap_real  mask(last_tap_real){BitWidthIn=14, CoeffBitWidth=18, mult_latency=2, use_hdl=on, use_embedded=off}
      mask prompts: BitWidthIn "Input Bitwidth:"; CoeffBitWidth "Coeff Bitwidth:"; mult_latency "Mult Latency"; use_hdl "Use behavioral HDL for multlipliers"; use_embedded "Use embedded multipliers"
      mask init:
      | last_tap_real_init(gcb,...
      |     'BitWidthIn', BitWidthIn,...
      |     'CoeffBitWidth', CoeffBitWidth,...
      |     'mult_latency', mult_latency,...
      |     'use_hdl', use_hdl,...
      |     'use_embedded', use_embedded);
      mask Callback use_hdl:
      | use_hdl = get_param(gcb,'use_hdl');
      | if( strcmp(use_hdl,'on')),
      |     set_param(gcb, 'use_embedded','off');
      |     set_param(gcb, 'MaskVisibilities',{'on','on','on','on','off'});
      | else,
      |     set_param(gcb, 'MaskVisibilities',{'on','on','on','on','on'});
      | end
  pol1_in5_tap2 : Subsystem  AncestorBlock=casper_library_pfbs/tap_real  mask(pfb_tap_real){mult_latency=2, coeff_width=18, coeff_frac_width=17, delay=2048, data_width=14, bram_latency=2, use_hdl=on, use_embedded=off}
      mask prompts: mult_latency "Multiplier Latency"; coeff_width "Coefficient Bit Width In"; coeff_frac_width "Coefficient Fractional Bits"; delay "Data/Sync Delay"; data_width "Data Bit Width In"; bram_latency "BRAM Latency"; use_hdl "Use behavioral HDL for multlipliers"; use_embedded "Use embedded multipliers"
      mask init: same as pfb_fft_d3a/pfb_fir_real/pol1_in1_tap2
  pol1_in5_tap3 : Subsystem  AncestorBlock=casper_library_pfbs/tap_real  mask(pfb_tap_real){mult_latency=2, coeff_width=18, coeff_frac_width=17, delay=2048, data_width=14, bram_latency=2, use_hdl=on, use_embedded=off}
      mask prompts: mult_latency "Multiplier Latency"; coeff_width "Coefficient Bit Width In"; coeff_frac_width "Coefficient Fractional Bits"; delay "Data/Sync Delay"; data_width "Data Bit Width In"; bram_latency "BRAM Latency"; use_hdl "Use behavioral HDL for multlipliers"; use_embedded "Use embedded multipliers"
      mask init: same as pfb_fft_d3a/pfb_fir_real/pol1_in1_tap2
  pol1_in6_coeffs : Subsystem  AncestorBlock=casper_library_pfbs/pfb_coeff_gen  mask(pfb_coeff_gen){PFBSize=14, CoeffBitWidth=18, TotalTaps=4, CoeffDistMem=off, WindowType=hamming, bram_latency=2, n_inputs=3, nput=5, fwidth=1, debug_mode=off, fan_latency=1}
      mask prompts: PFBSize "Size of PFB: (2^? pnts)"; CoeffBitWidth "Bitwidth of Coefficients:"; TotalTaps "Total Number of Taps:"; CoeffDistMem "Implement Coeff Gen in Distributed Memory"; WindowType "Windowing Function:"; bram_latency "BRAM Latency"; n_inputs "Number of Simultaneous Inputs: (2^?)"; nput "This is input number:"; fwidth "Bin Width (normal=1)"; debug_mode "Debug mode - coeffs are a [1:pfb_size*taps] ramp."; fan_latency "Fanout latency"
      mask init: same as pfb_fft_d3a/pfb_fir_real/pol1_in1_coeffs
      settings: AttributesFormatString=|
      | PFBSize=14, n_inputs=3,
      | taps=4, input=5
  pol1_in6_first_tap : Subsystem  AncestorBlock=casper_library_pfbs/first_tap_real  mask(first_tap_real){PFBSize=14, n_pol_blocks=1, CoeffBitWidth=18, TotalTaps=4, BitWidthIn=14, WindowType=hamming, mult_latency=2, bram_latency=2, n_inputs=3, fwidth=1, use_hdl=on, use_embedded=off}
      mask prompts: PFBSize "Size of PFB: (2^? pnts)"; n_pol_blocks "Number of serial polarization blocks"; CoeffBitWidth "Bitwidth of Coefficients:"; TotalTaps "Total Number of Taps:"; BitWidthIn "Input Bitwidth:"; WindowType "Windowing Function:"; mult_latency "Mult Latency"; bram_latency "BRAM Latency"; n_inputs "Number of Simultaneous Inputs: (2^?)"; fwidth "Bit Width (normal=1)"; use_hdl "Use behavioral HDL for multlipliers"; use_embedded "Use embedded multipliers"
      mask init: same as pfb_fft_d3a/pfb_fir_real/pol1_in1_first_tap
      settings: AttributesFormatString=taps=4
      mask TypeOptions WindowType: bartlett | barthannwin | blackman | blackmanharris | bohamwin | chebwin | flattopwin | gausswin | hamming | hann | kaiser | nuttallwin | parzenwin | rectwin | tukeywin | triang | userwindow
      mask Callback use_hdl:
      | use_hdl = get_param(gcb,'use_hdl');
      | if( strcmp(use_hdl,'on')),
      |     set_param(gcb, 'use_embedded','off');
      |     set_param(gcb, 'MaskVisibilities',{'on','on','on','on','on','on','on','on','on','on','on','off'});
      | else,
      |     set_param(gcb, 'MaskVisibilities',{'on','on','on','on','on','on','on','on','on','on','on','on'});
      | end
  pol1_in6_last_tap : Subsystem  AncestorBlock=casper_library_pfbs/last_tap_real  mask(last_tap_real){BitWidthIn=14, CoeffBitWidth=18, mult_latency=2, use_hdl=on, use_embedded=off}
      mask prompts: BitWidthIn "Input Bitwidth:"; CoeffBitWidth "Coeff Bitwidth:"; mult_latency "Mult Latency"; use_hdl "Use behavioral HDL for multlipliers"; use_embedded "Use embedded multipliers"
      mask init:
      | last_tap_real_init(gcb,...
      |     'BitWidthIn', BitWidthIn,...
      |     'CoeffBitWidth', CoeffBitWidth,...
      |     'mult_latency', mult_latency,...
      |     'use_hdl', use_hdl,...
      |     'use_embedded', use_embedded);
      mask Callback use_hdl:
      | use_hdl = get_param(gcb,'use_hdl');
      | if( strcmp(use_hdl,'on')),
      |     set_param(gcb, 'use_embedded','off');
      |     set_param(gcb, 'MaskVisibilities',{'on','on','on','on','off'});
      | else,
      |     set_param(gcb, 'MaskVisibilities',{'on','on','on','on','on'});
      | end
  pol1_in6_tap2 : Subsystem  AncestorBlock=casper_library_pfbs/tap_real  mask(pfb_tap_real){mult_latency=2, coeff_width=18, coeff_frac_width=17, delay=2048, data_width=14, bram_latency=2, use_hdl=on, use_embedded=off}
      mask prompts: mult_latency "Multiplier Latency"; coeff_width "Coefficient Bit Width In"; coeff_frac_width "Coefficient Fractional Bits"; delay "Data/Sync Delay"; data_width "Data Bit Width In"; bram_latency "BRAM Latency"; use_hdl "Use behavioral HDL for multlipliers"; use_embedded "Use embedded multipliers"
      mask init: same as pfb_fft_d3a/pfb_fir_real/pol1_in1_tap2
  pol1_in6_tap3 : Subsystem  AncestorBlock=casper_library_pfbs/tap_real  mask(pfb_tap_real){mult_latency=2, coeff_width=18, coeff_frac_width=17, delay=2048, data_width=14, bram_latency=2, use_hdl=on, use_embedded=off}
      mask prompts: mult_latency "Multiplier Latency"; coeff_width "Coefficient Bit Width In"; coeff_frac_width "Coefficient Fractional Bits"; delay "Data/Sync Delay"; data_width "Data Bit Width In"; bram_latency "BRAM Latency"; use_hdl "Use behavioral HDL for multlipliers"; use_embedded "Use embedded multipliers"
      mask init: same as pfb_fft_d3a/pfb_fir_real/pol1_in1_tap2
  pol1_in7_coeffs : Subsystem  AncestorBlock=casper_library_pfbs/pfb_coeff_gen  mask(pfb_coeff_gen){PFBSize=14, CoeffBitWidth=18, TotalTaps=4, CoeffDistMem=off, WindowType=hamming, bram_latency=2, n_inputs=3, nput=6, fwidth=1, debug_mode=off, fan_latency=1}
      mask prompts: PFBSize "Size of PFB: (2^? pnts)"; CoeffBitWidth "Bitwidth of Coefficients:"; TotalTaps "Total Number of Taps:"; CoeffDistMem "Implement Coeff Gen in Distributed Memory"; WindowType "Windowing Function:"; bram_latency "BRAM Latency"; n_inputs "Number of Simultaneous Inputs: (2^?)"; nput "This is input number:"; fwidth "Bin Width (normal=1)"; debug_mode "Debug mode - coeffs are a [1:pfb_size*taps] ramp."; fan_latency "Fanout latency"
      mask init: same as pfb_fft_d3a/pfb_fir_real/pol1_in1_coeffs
      settings: AttributesFormatString=|
      | PFBSize=14, n_inputs=3,
      | taps=4, input=6
  pol1_in7_first_tap : Subsystem  AncestorBlock=casper_library_pfbs/first_tap_real  mask(first_tap_real){PFBSize=14, n_pol_blocks=1, CoeffBitWidth=18, TotalTaps=4, BitWidthIn=14, WindowType=hamming, mult_latency=2, bram_latency=2, n_inputs=3, fwidth=1, use_hdl=on, use_embedded=off}
      mask prompts: PFBSize "Size of PFB: (2^? pnts)"; n_pol_blocks "Number of serial polarization blocks"; CoeffBitWidth "Bitwidth of Coefficients:"; TotalTaps "Total Number of Taps:"; BitWidthIn "Input Bitwidth:"; WindowType "Windowing Function:"; mult_latency "Mult Latency"; bram_latency "BRAM Latency"; n_inputs "Number of Simultaneous Inputs: (2^?)"; fwidth "Bit Width (normal=1)"; use_hdl "Use behavioral HDL for multlipliers"; use_embedded "Use embedded multipliers"
      mask init: same as pfb_fft_d3a/pfb_fir_real/pol1_in1_first_tap
      settings: AttributesFormatString=taps=4
      mask TypeOptions WindowType: bartlett | barthannwin | blackman | blackmanharris | bohamwin | chebwin | flattopwin | gausswin | hamming | hann | kaiser | nuttallwin | parzenwin | rectwin | tukeywin | triang | userwindow
      mask Callback use_hdl:
      | use_hdl = get_param(gcb,'use_hdl');
      | if( strcmp(use_hdl,'on')),
      |     set_param(gcb, 'use_embedded','off');
      |     set_param(gcb, 'MaskVisibilities',{'on','on','on','on','on','on','on','on','on','on','on','off'});
      | else,
      |     set_param(gcb, 'MaskVisibilities',{'on','on','on','on','on','on','on','on','on','on','on','on'});
      | end
  pol1_in7_last_tap : Subsystem  AncestorBlock=casper_library_pfbs/last_tap_real  mask(last_tap_real){BitWidthIn=14, CoeffBitWidth=18, mult_latency=2, use_hdl=on, use_embedded=off}
      mask prompts: BitWidthIn "Input Bitwidth:"; CoeffBitWidth "Coeff Bitwidth:"; mult_latency "Mult Latency"; use_hdl "Use behavioral HDL for multlipliers"; use_embedded "Use embedded multipliers"
      mask init:
      | last_tap_real_init(gcb,...
      |     'BitWidthIn', BitWidthIn,...
      |     'CoeffBitWidth', CoeffBitWidth,...
      |     'mult_latency', mult_latency,...
      |     'use_hdl', use_hdl,...
      |     'use_embedded', use_embedded);
      mask Callback use_hdl:
      | use_hdl = get_param(gcb,'use_hdl');
      | if( strcmp(use_hdl,'on')),
      |     set_param(gcb, 'use_embedded','off');
      |     set_param(gcb, 'MaskVisibilities',{'on','on','on','on','off'});
      | else,
      |     set_param(gcb, 'MaskVisibilities',{'on','on','on','on','on'});
      | end
  pol1_in7_tap2 : Subsystem  AncestorBlock=casper_library_pfbs/tap_real  mask(pfb_tap_real){mult_latency=2, coeff_width=18, coeff_frac_width=17, delay=2048, data_width=14, bram_latency=2, use_hdl=on, use_embedded=off}
      mask prompts: mult_latency "Multiplier Latency"; coeff_width "Coefficient Bit Width In"; coeff_frac_width "Coefficient Fractional Bits"; delay "Data/Sync Delay"; data_width "Data Bit Width In"; bram_latency "BRAM Latency"; use_hdl "Use behavioral HDL for multlipliers"; use_embedded "Use embedded multipliers"
      mask init: same as pfb_fft_d3a/pfb_fir_real/pol1_in1_tap2
  pol1_in7_tap3 : Subsystem  AncestorBlock=casper_library_pfbs/tap_real  mask(pfb_tap_real){mult_latency=2, coeff_width=18, coeff_frac_width=17, delay=2048, data_width=14, bram_latency=2, use_hdl=on, use_embedded=off}
      mask prompts: mult_latency "Multiplier Latency"; coeff_width "Coefficient Bit Width In"; coeff_frac_width "Coefficient Fractional Bits"; delay "Data/Sync Delay"; data_width "Data Bit Width In"; bram_latency "BRAM Latency"; use_hdl "Use behavioral HDL for multlipliers"; use_embedded "Use embedded multipliers"
      mask init: same as pfb_fft_d3a/pfb_fir_real/pol1_in1_tap2
  pol1_in8_coeffs : Subsystem  AncestorBlock=casper_library_pfbs/pfb_coeff_gen  mask(pfb_coeff_gen){PFBSize=14, CoeffBitWidth=18, TotalTaps=4, CoeffDistMem=off, WindowType=hamming, bram_latency=2, n_inputs=3, nput=7, fwidth=1, debug_mode=off, fan_latency=1}
      mask prompts: PFBSize "Size of PFB: (2^? pnts)"; CoeffBitWidth "Bitwidth of Coefficients:"; TotalTaps "Total Number of Taps:"; CoeffDistMem "Implement Coeff Gen in Distributed Memory"; WindowType "Windowing Function:"; bram_latency "BRAM Latency"; n_inputs "Number of Simultaneous Inputs: (2^?)"; nput "This is input number:"; fwidth "Bin Width (normal=1)"; debug_mode "Debug mode - coeffs are a [1:pfb_size*taps] ramp."; fan_latency "Fanout latency"
      mask init: same as pfb_fft_d3a/pfb_fir_real/pol1_in1_coeffs
      settings: AttributesFormatString=|
      | PFBSize=14, n_inputs=3,
      | taps=4, input=7
  pol1_in8_first_tap : Subsystem  AncestorBlock=casper_library_pfbs/first_tap_real  mask(first_tap_real){PFBSize=14, n_pol_blocks=1, CoeffBitWidth=18, TotalTaps=4, BitWidthIn=14, WindowType=hamming, mult_latency=2, bram_latency=2, n_inputs=3, fwidth=1, use_hdl=on, use_embedded=off}
      mask prompts: PFBSize "Size of PFB: (2^? pnts)"; n_pol_blocks "Number of serial polarization blocks"; CoeffBitWidth "Bitwidth of Coefficients:"; TotalTaps "Total Number of Taps:"; BitWidthIn "Input Bitwidth:"; WindowType "Windowing Function:"; mult_latency "Mult Latency"; bram_latency "BRAM Latency"; n_inputs "Number of Simultaneous Inputs: (2^?)"; fwidth "Bit Width (normal=1)"; use_hdl "Use behavioral HDL for multlipliers"; use_embedded "Use embedded multipliers"
      mask init: same as pfb_fft_d3a/pfb_fir_real/pol1_in1_first_tap
      settings: AttributesFormatString=taps=4
      mask TypeOptions WindowType: bartlett | barthannwin | blackman | blackmanharris | bohamwin | chebwin | flattopwin | gausswin | hamming | hann | kaiser | nuttallwin | parzenwin | rectwin | tukeywin | triang | userwindow
      mask Callback use_hdl:
      | use_hdl = get_param(gcb,'use_hdl');
      | if( strcmp(use_hdl,'on')),
      |     set_param(gcb, 'use_embedded','off');
      |     set_param(gcb, 'MaskVisibilities',{'on','on','on','on','on','on','on','on','on','on','on','off'});
      | else,
      |     set_param(gcb, 'MaskVisibilities',{'on','on','on','on','on','on','on','on','on','on','on','on'});
      | end
  pol1_in8_last_tap : Subsystem  AncestorBlock=casper_library_pfbs/last_tap_real  mask(last_tap_real){BitWidthIn=14, CoeffBitWidth=18, mult_latency=2, use_hdl=on, use_embedded=off}
      mask prompts: BitWidthIn "Input Bitwidth:"; CoeffBitWidth "Coeff Bitwidth:"; mult_latency "Mult Latency"; use_hdl "Use behavioral HDL for multlipliers"; use_embedded "Use embedded multipliers"
      mask init:
      | last_tap_real_init(gcb,...
      |     'BitWidthIn', BitWidthIn,...
      |     'CoeffBitWidth', CoeffBitWidth,...
      |     'mult_latency', mult_latency,...
      |     'use_hdl', use_hdl,...
      |     'use_embedded', use_embedded);
      mask Callback use_hdl:
      | use_hdl = get_param(gcb,'use_hdl');
      | if( strcmp(use_hdl,'on')),
      |     set_param(gcb, 'use_embedded','off');
      |     set_param(gcb, 'MaskVisibilities',{'on','on','on','on','off'});
      | else,
      |     set_param(gcb, 'MaskVisibilities',{'on','on','on','on','on'});
      | end
  pol1_in8_tap2 : Subsystem  AncestorBlock=casper_library_pfbs/tap_real  mask(pfb_tap_real){mult_latency=2, coeff_width=18, coeff_frac_width=17, delay=2048, data_width=14, bram_latency=2, use_hdl=on, use_embedded=off}
      mask prompts: mult_latency "Multiplier Latency"; coeff_width "Coefficient Bit Width In"; coeff_frac_width "Coefficient Fractional Bits"; delay "Data/Sync Delay"; data_width "Data Bit Width In"; bram_latency "BRAM Latency"; use_hdl "Use behavioral HDL for multlipliers"; use_embedded "Use embedded multipliers"
      mask init: same as pfb_fft_d3a/pfb_fir_real/pol1_in1_tap2
  pol1_in8_tap3 : Subsystem  AncestorBlock=casper_library_pfbs/tap_real  mask(pfb_tap_real){mult_latency=2, coeff_width=18, coeff_frac_width=17, delay=2048, data_width=14, bram_latency=2, use_hdl=on, use_embedded=off}
      mask prompts: mult_latency "Multiplier Latency"; coeff_width "Coefficient Bit Width In"; coeff_frac_width "Coefficient Fractional Bits"; delay "Data/Sync Delay"; data_width "Data Bit Width In"; bram_latency "BRAM Latency"; use_hdl "Use behavioral HDL for multlipliers"; use_embedded "Use embedded multipliers"
      mask init: same as pfb_fft_d3a/pfb_fir_real/pol1_in1_tap2
  scale_1_{1..8} (8 alike) : xbsIndex_r4/Scale  scale_factor=-1  dbl_ovrd=off  block_type=scale
  sync_out : Outport  VectorParamsAs1DForOutWhenUnconnected=off
  pol1_out1 : Outport  Port=2  VectorParamsAs1DForOutWhenUnconnected=off
  pol1_out2 : Outport  Port=3  VectorParamsAs1DForOutWhenUnconnected=off
  pol1_out3 : Outport  Port=4
  pol1_out4 : Outport  Port=5
  pol1_out5 : Outport  Port=6
  pol1_out6 : Outport  Port=7
  pol1_out7 : Outport  Port=8
  pol1_out8 : Outport  Port=9
  wires:
  pol1_in1/1 -> pol1_in1_coeffs/1(din)
  sync/1 -> pol1_in1_coeffs/2(sync), pol1_in2_coeffs/2(sync), pol1_in3_coeffs/2(sync), pol1_in4_coeffs/2(sync), pol1_in5_coeffs/2(sync), pol1_in6_coeffs/2(sync), pol1_in7_coeffs/2(sync), pol1_in8_coeffs/2(sync)
  pol1_in1_coeffs/1(dout) -> pol1_in1_first_tap/1(din)
  pol1_in1_coeffs/2(sync_out) -> pol1_in1_first_tap/2(sync), pol1_in2_first_tap/2(sync), pol1_in3_first_tap/2(sync), pol1_in4_first_tap/2(sync), pol1_in5_first_tap/2(sync), pol1_in6_first_tap/2(sync), pol1_in7_first_tap/2(sync), pol1_in8_first_tap/2(sync)
  pol1_in1_coeffs/3(coeff) -> pol1_in1_first_tap/3(coeffs)
  pol1_in2/1 -> pol1_in2_coeffs/1(din)
  pol1_in2_coeffs/1(dout) -> pol1_in2_first_tap/1(din)
  pol1_in2_coeffs/3(coeff) -> pol1_in2_first_tap/3(coeffs)
  pol1_in3/1 -> pol1_in3_coeffs/1(din)
  pol1_in3_coeffs/1(dout) -> pol1_in3_first_tap/1(din)
  pol1_in3_coeffs/3(coeff) -> pol1_in3_first_tap/3(coeffs)
  pol1_in4/1 -> pol1_in4_coeffs/1(din)
  pol1_in4_coeffs/1(dout) -> pol1_in4_first_tap/1(din)
  pol1_in4_coeffs/3(coeff) -> pol1_in4_first_tap/3(coeffs)
  pol1_in5/1 -> pol1_in5_coeffs/1(din)
  pol1_in5_coeffs/1(dout) -> pol1_in5_first_tap/1(din)
  pol1_in5_coeffs/3(coeff) -> pol1_in5_first_tap/3(coeffs)
  pol1_in6/1 -> pol1_in6_coeffs/1(din)
  pol1_in6_coeffs/1(dout) -> pol1_in6_first_tap/1(din)
  pol1_in6_coeffs/3(coeff) -> pol1_in6_first_tap/3(coeffs)
  pol1_in7/1 -> pol1_in7_coeffs/1(din)
  pol1_in7_coeffs/1(dout) -> pol1_in7_first_tap/1(din)
  pol1_in7_coeffs/3(coeff) -> pol1_in7_first_tap/3(coeffs)
  pol1_in8/1 -> pol1_in8_coeffs/1(din)
  pol1_in8_coeffs/1(dout) -> pol1_in8_first_tap/1(din)
  pol1_in8_coeffs/3(coeff) -> pol1_in8_first_tap/3(coeffs)
  adder_1_1/1(sync_out) -> delay1/1
  delay1/1 -> sync_out/1
  adder_1_1/2(dout) -> scale_1_1/1
  scale_1_1/1 -> convert_1_1/1
  convert_1_1/1 -> pol1_out1/1
  adder_1_2/2(dout) -> scale_1_2/1
  scale_1_2/1 -> convert_1_2/1
  convert_1_2/1 -> pol1_out2/1
  adder_1_3/2(dout) -> scale_1_3/1
  scale_1_3/1 -> convert_1_3/1
  convert_1_3/1 -> pol1_out3/1
  adder_1_4/2(dout) -> scale_1_4/1
  scale_1_4/1 -> convert_1_4/1
  convert_1_4/1 -> pol1_out4/1
  adder_1_5/2(dout) -> scale_1_5/1
  scale_1_5/1 -> convert_1_5/1
  convert_1_5/1 -> pol1_out5/1
  adder_1_6/2(dout) -> scale_1_6/1
  scale_1_6/1 -> convert_1_6/1
  convert_1_6/1 -> pol1_out6/1
  adder_1_7/2(dout) -> scale_1_7/1
  scale_1_7/1 -> convert_1_7/1
  convert_1_7/1 -> pol1_out7/1
  adder_1_8/2(dout) -> scale_1_8/1
  scale_1_8/1 -> convert_1_8/1
  convert_1_8/1 -> pol1_out8/1
  pol1_in1_first_tap/1(dout) -> pol1_in1_tap2/1(din)
  pol1_in1_first_tap/2(sync_out) -> pol1_in1_tap2/2(sync)
  pol1_in1_first_tap/3(coeff_out) -> pol1_in1_tap2/3(coeff)
  pol1_in1_first_tap/4(taps_out) -> adder_1_1/2(din1)
  pol1_in1_tap2/1(dout) -> pol1_in1_tap3/1(din)
  pol1_in1_tap2/2(sync_out) -> pol1_in1_tap3/2(sync)
  pol1_in1_tap2/3(coeff_out) -> pol1_in1_tap3/3(coeff)
  pol1_in1_tap2/4(taps_out) -> adder_1_1/3(din2)
  pol1_in1_last_tap/2(sync_out) -> adder_1_1/1(sync)
  pol1_in1_last_tap/1(tap_out) -> adder_1_1/5(din4)
  pol1_in1_tap3/1(dout) -> pol1_in1_last_tap/1(din)
  pol1_in1_tap3/2(sync_out) -> pol1_in1_last_tap/2(sync)
  pol1_in1_tap3/3(coeff_out) -> pol1_in1_last_tap/3(coeff)
  pol1_in1_tap3/4(taps_out) -> adder_1_1/4(din3)
  pol1_in2_first_tap/1(dout) -> pol1_in2_tap2/1(din)
  pol1_in2_first_tap/2(sync_out) -> pol1_in2_tap2/2(sync)
  pol1_in2_first_tap/3(coeff_out) -> pol1_in2_tap2/3(coeff)
  pol1_in2_first_tap/4(taps_out) -> adder_1_2/2(din1)
  pol1_in2_tap2/1(dout) -> pol1_in2_tap3/1(din)
  pol1_in2_tap2/2(sync_out) -> pol1_in2_tap3/2(sync)
  pol1_in2_tap2/3(coeff_out) -> pol1_in2_tap3/3(coeff)
  pol1_in2_tap2/4(taps_out) -> adder_1_2/3(din2)
  pol1_in2_last_tap/2(sync_out) -> adder_1_2/1(sync)
  pol1_in2_last_tap/1(tap_out) -> adder_1_2/5(din4)
  pol1_in2_tap3/1(dout) -> pol1_in2_last_tap/1(din)
  pol1_in2_tap3/2(sync_out) -> pol1_in2_last_tap/2(sync)
  pol1_in2_tap3/3(coeff_out) -> pol1_in2_last_tap/3(coeff)
  pol1_in2_tap3/4(taps_out) -> adder_1_2/4(din3)
  pol1_in3_first_tap/1(dout) -> pol1_in3_tap2/1(din)
  pol1_in3_first_tap/2(sync_out) -> pol1_in3_tap2/2(sync)
  pol1_in3_first_tap/3(coeff_out) -> pol1_in3_tap2/3(coeff)
  pol1_in3_first_tap/4(taps_out) -> adder_1_3/2(din1)
  pol1_in3_tap2/1(dout) -> pol1_in3_tap3/1(din)
  pol1_in3_tap2/2(sync_out) -> pol1_in3_tap3/2(sync)
  pol1_in3_tap2/3(coeff_out) -> pol1_in3_tap3/3(coeff)
  pol1_in3_tap2/4(taps_out) -> adder_1_3/3(din2)
  pol1_in3_last_tap/2(sync_out) -> adder_1_3/1(sync)
  pol1_in3_last_tap/1(tap_out) -> adder_1_3/5(din4)
  pol1_in3_tap3/1(dout) -> pol1_in3_last_tap/1(din)
  pol1_in3_tap3/2(sync_out) -> pol1_in3_last_tap/2(sync)
  pol1_in3_tap3/3(coeff_out) -> pol1_in3_last_tap/3(coeff)
  pol1_in3_tap3/4(taps_out) -> adder_1_3/4(din3)
  pol1_in4_first_tap/1(dout) -> pol1_in4_tap2/1(din)
  pol1_in4_first_tap/2(sync_out) -> pol1_in4_tap2/2(sync)
  pol1_in4_first_tap/3(coeff_out) -> pol1_in4_tap2/3(coeff)
  pol1_in4_first_tap/4(taps_out) -> adder_1_4/2(din1)
  pol1_in4_tap2/1(dout) -> pol1_in4_tap3/1(din)
  pol1_in4_tap2/2(sync_out) -> pol1_in4_tap3/2(sync)
  pol1_in4_tap2/3(coeff_out) -> pol1_in4_tap3/3(coeff)
  pol1_in4_tap2/4(taps_out) -> adder_1_4/3(din2)
  pol1_in4_last_tap/2(sync_out) -> adder_1_4/1(sync)
  pol1_in4_last_tap/1(tap_out) -> adder_1_4/5(din4)
  pol1_in4_tap3/1(dout) -> pol1_in4_last_tap/1(din)
  pol1_in4_tap3/2(sync_out) -> pol1_in4_last_tap/2(sync)
  pol1_in4_tap3/3(coeff_out) -> pol1_in4_last_tap/3(coeff)
  pol1_in4_tap3/4(taps_out) -> adder_1_4/4(din3)
  pol1_in5_first_tap/1(dout) -> pol1_in5_tap2/1(din)
  pol1_in5_first_tap/2(sync_out) -> pol1_in5_tap2/2(sync)
  pol1_in5_first_tap/3(coeff_out) -> pol1_in5_tap2/3(coeff)
  pol1_in5_first_tap/4(taps_out) -> adder_1_5/2(din1)
  pol1_in5_tap2/1(dout) -> pol1_in5_tap3/1(din)
  pol1_in5_tap2/2(sync_out) -> pol1_in5_tap3/2(sync)
  pol1_in5_tap2/3(coeff_out) -> pol1_in5_tap3/3(coeff)
  pol1_in5_tap2/4(taps_out) -> adder_1_5/3(din2)
  pol1_in5_last_tap/2(sync_out) -> adder_1_5/1(sync)
  pol1_in5_last_tap/1(tap_out) -> adder_1_5/5(din4)
  pol1_in5_tap3/1(dout) -> pol1_in5_last_tap/1(din)
  pol1_in5_tap3/2(sync_out) -> pol1_in5_last_tap/2(sync)
  pol1_in5_tap3/3(coeff_out) -> pol1_in5_last_tap/3(coeff)
  pol1_in5_tap3/4(taps_out) -> adder_1_5/4(din3)
  pol1_in6_first_tap/1(dout) -> pol1_in6_tap2/1(din)
  pol1_in6_first_tap/2(sync_out) -> pol1_in6_tap2/2(sync)
  pol1_in6_first_tap/3(coeff_out) -> pol1_in6_tap2/3(coeff)
  pol1_in6_first_tap/4(taps_out) -> adder_1_6/2(din1)
  pol1_in6_tap2/1(dout) -> pol1_in6_tap3/1(din)
  pol1_in6_tap2/2(sync_out) -> pol1_in6_tap3/2(sync)
  pol1_in6_tap2/3(coeff_out) -> pol1_in6_tap3/3(coeff)
  pol1_in6_tap2/4(taps_out) -> adder_1_6/3(din2)
  pol1_in6_last_tap/2(sync_out) -> adder_1_6/1(sync)
  pol1_in6_last_tap/1(tap_out) -> adder_1_6/5(din4)
  pol1_in6_tap3/1(dout) -> pol1_in6_last_tap/1(din)
  pol1_in6_tap3/2(sync_out) -> pol1_in6_last_tap/2(sync)
  pol1_in6_tap3/3(coeff_out) -> pol1_in6_last_tap/3(coeff)
  pol1_in6_tap3/4(taps_out) -> adder_1_6/4(din3)
  pol1_in7_first_tap/1(dout) -> pol1_in7_tap2/1(din)
  pol1_in7_first_tap/2(sync_out) -> pol1_in7_tap2/2(sync)
  pol1_in7_first_tap/3(coeff_out) -> pol1_in7_tap2/3(coeff)
  pol1_in7_first_tap/4(taps_out) -> adder_1_7/2(din1)
  pol1_in7_tap2/1(dout) -> pol1_in7_tap3/1(din)
  pol1_in7_tap2/2(sync_out) -> pol1_in7_tap3/2(sync)
  pol1_in7_tap2/3(coeff_out) -> pol1_in7_tap3/3(coeff)
  pol1_in7_tap2/4(taps_out) -> adder_1_7/3(din2)
  pol1_in7_last_tap/2(sync_out) -> adder_1_7/1(sync)
  pol1_in7_last_tap/1(tap_out) -> adder_1_7/5(din4)
  pol1_in7_tap3/1(dout) -> pol1_in7_last_tap/1(din)
  pol1_in7_tap3/2(sync_out) -> pol1_in7_last_tap/2(sync)
  pol1_in7_tap3/3(coeff_out) -> pol1_in7_last_tap/3(coeff)
  pol1_in7_tap3/4(taps_out) -> adder_1_7/4(din3)
  pol1_in8_first_tap/1(dout) -> pol1_in8_tap2/1(din)
  pol1_in8_first_tap/2(sync_out) -> pol1_in8_tap2/2(sync)
  pol1_in8_first_tap/3(coeff_out) -> pol1_in8_tap2/3(coeff)
  pol1_in8_first_tap/4(taps_out) -> adder_1_8/2(din1)
  pol1_in8_tap2/1(dout) -> pol1_in8_tap3/1(din)
  pol1_in8_tap2/2(sync_out) -> pol1_in8_tap3/2(sync)
  pol1_in8_tap2/3(coeff_out) -> pol1_in8_tap3/3(coeff)
  pol1_in8_tap2/4(taps_out) -> adder_1_8/3(din2)
  pol1_in8_last_tap/2(sync_out) -> adder_1_8/1(sync)
  pol1_in8_last_tap/1(tap_out) -> adder_1_8/5(din4)
  pol1_in8_tap3/1(dout) -> pol1_in8_last_tap/1(din)
  pol1_in8_tap3/2(sync_out) -> pol1_in8_last_tap/2(sync)
  pol1_in8_tap3/3(coeff_out) -> pol1_in8_last_tap/3(coeff)
  pol1_in8_tap3/4(taps_out) -> adder_1_8/4(din3)
